simulink model "led"  (R2025b)
settings: Solver=VariableStepAuto  StartTime=0.0  StopTime=10.0  RelTol=1e-3
libraries: arduinolib x1, simulink x1
settings Model: Creator=00782620  LastModifiedBy=00782620

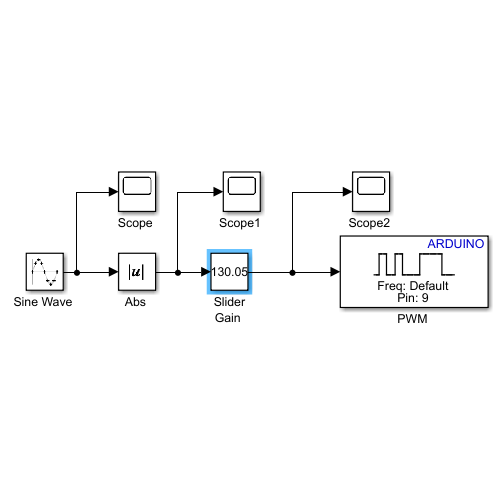
[thumbnail: Simulink's stored preview of the top-level diagram]
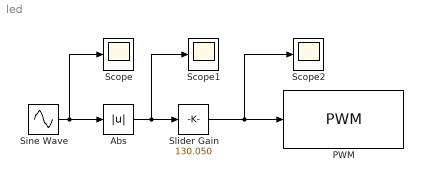
== system led ==
  "Abs " : Abs  SaturateOnIntegerOverflow=off
  "PWM " : arduinolib/PWM  pinNumber=9  frequencyType=Default  desiredFrequency=490.2  achievableFrequency=490.2
  "Scope " : Scope
  "Scope1 " : Scope
  "Scope2 " : Scope
      settings: DataLoggingVariableName=ScopeData2
  "Sine Wave " : Sin  SineType=Sample based  Samples=300  SampleTime=0.01
  "Slider Gain " : simulink/Math Operations/Slider Gain  gain=130.050  low=0  high=255
  wires:
  "Sine Wave "/1 -> "Scope "/1, "Abs "/1
  "Abs "/1 -> "Slider Gain "/1, "Scope1 "/1
  "Slider Gain "/1 -> "Scope2 "/1, "PWM "/1
